simulink model "TAFC5B01"  (R2025b)
settings: Solver=ode4  StartTime=0.0  StopTime=inf  FixedStep=0.002  RelTol=1e-3
undefined symbols (not defined in the file): RS232, RS422, TTL, UART4, UART5, UART6, UART7, UART8
libraries: AFCToolbox x62, AFC5Toolbox x12, etargetslib x10, simulink x5
settings Model: Creator=Administrator  LastModifiedBy=zqhkd
settings OptimizationCC: DefaultParameterBehavior=Inlined  EnhancedBackFolding=on  PassReuseOutputArgsAs=Individual arguments  ZeroExternalMemoryAtStartup=off  ZeroInternalMemoryAtStartup=off  OptimizeBlockOrder=speed  DifferentSizesBufferReuse=on  OptimizationCustomize=off  EfficientTunableParamExpr=on
settings DebuggingCC: ParameterPrecisionLossMsg=none  ParameterTunabilityLossMsg=error
settings HardwareCC: ProdBitPerInt=16.0  ProdBitPerPointer=16.0  ProdBitPerSizeT=16.0  ProdBitPerPtrDiffT=16.0  ProdLargestAtomicFloat=None  ProdWordSize=16.0  ProdHWDeviceType=STMicroelectronics->ST10/Super10
settings SFSimCC: MATLABDynamicMemAlloc=off
settings RTWCC: SystemTargetFile=AFCHawk.tlc  GenCodeOnly=on  TemplateMakefile=ert_default_tmf  GPUComputeCapability=3.5  Description=Embedded Coder
settings CodeAppCC: ForceParamTrailComments=on  IgnoreCustomStorageClasses=off  OperatorAnnotations=on  SimulinkDataObjDesc=on  SFDataObjDesc=on  InsertBlockDesc=on
settings STFCustomTargetCC: SystemTargetFile=AFCHawk.tlc  TargetLangStandard=C99 (ISO)  MultiwordLength=256.0  ModelReferenceCompliant=off  ConcurrentExecutionCompliant=off  CombineOutputUpdateFcns=on  ERTCustomFileBanners=on  SupportContinuousTime=off  SupportNonInlinedSFcns=off  RemoveResetFunc=on  MATLABClassNameForMDSCustomization=Simulink.SoftwareTarget.ERTCustomization  GRTInterface=off  t_comBaud=460800.0  t_comPort=2.0  t_BuildCPrj2Hex=on  t_DownLoad2Target=on
settings ERTTargetCC: ERTCustomFileTemplate=example_file_process.tlc  DynamicArrayContainerType=coder::array  TargetLangStandard=C99 (ISO)  ModelReferenceCompliant=off  ParMdlRefBuildCompliant=off  CompOptLevelCompliant=off  ConcurrentExecutionCompliant=off  ModelStepFunctionPrototypeControlCompliant=off  CPPClassGenCompliant=off  UseToolchainInfoCompliant=off

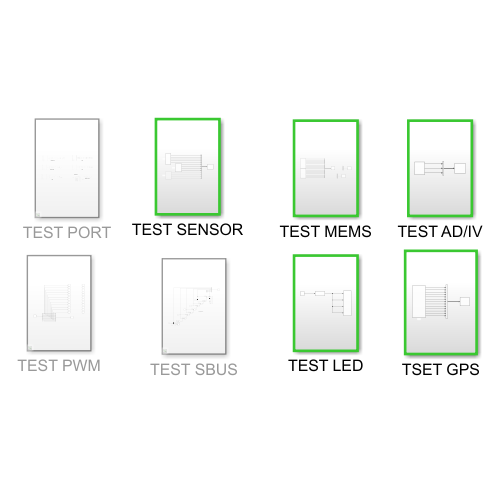
[thumbnail: Simulink's stored preview of the top-level diagram]
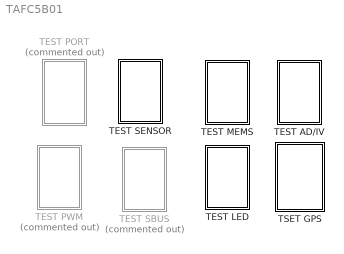
== system TAFC5B01 ==
  TEST AD/IV : Subsystem
  TEST LED : Subsystem
  TEST MEMS : Subsystem
  TEST PORT : Subsystem  Commented=on
  TEST PWM : Subsystem  Commented=on
  TEST SBUS : Subsystem  Commented=on
  TEST SENSOR : Subsystem
  TSET GPS : Subsystem

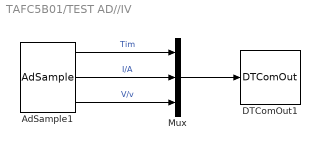
== system TAFC5B01/TEST AD//IV ==
  AdSample1 : AFCToolbox/DeviceModule/AdSample  Priority=1  g_sampleTime=0.01  g_comPort=0  g_instName=0  g_id=0
      settings: SourceProductName=AFCToolbox
  DTComOut1 : AFCToolbox/DeviceModule/DTComOut  Priority=8  g_frameType=12  g_outFreq=1  g_comPort=0  g_instName=0  g_id=0
      settings: SourceProductName=AFCToolbox
  Mux : Mux  Inputs=3
  wires:
  Mux/1 -> DTComOut1/1
  AdSample1/1 -> Mux/1  "Tim"
  AdSample1/2 -> Mux/2  "I/A"
  AdSample1/3 -> Mux/3  "V/v"

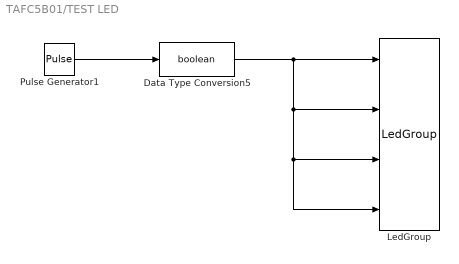
== system TAFC5B01/TEST LED ==
  Data Type Conversion5 : DataTypeConversion  OutDataTypeStr=boolean  SaturateOnIntegerOverflow=off  RndMeth=Floor
  LedGroup : AFCToolbox/DeviceModule/LedGroup  Priority=7  g_frameType=0  g_comPort=6  g_instName=0  g_id=0
      settings: SourceProductName=AFCToolbox
  Pulse Generator1 : DiscretePulseGenerator  Period=100  PulseWidth=50  SampleTime=0.01
  wires:
  Data Type Conversion5/1 -> LedGroup/2, LedGroup/4, LedGroup/3, LedGroup/1
  Pulse Generator1/1 -> Data Type Conversion5/1

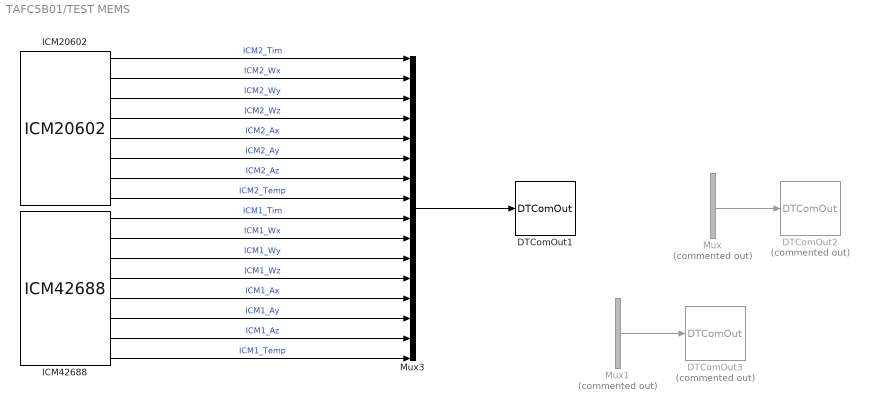
== system TAFC5B01/TEST MEMS ==
  DTComOut1 : AFCToolbox/DeviceModule/DTComOut  Priority=8  g_frameType=3  g_outFreq=10  g_comPort=0  g_instName=0  g_id=0
      settings: SourceProductName=AFCToolbox
  DTComOut2 : AFCToolbox/DeviceModule/DTComOut  Priority=8  Commented=on  g_frameType=1  g_outFreq=1  g_comPort=0  g_instName=0  g_id=0
      settings: SourceProductName=AFCToolbox
  DTComOut3 : AFCToolbox/DeviceModule/DTComOut  Priority=8  Commented=on  g_frameType=2  g_outFreq=1  g_comPort=0  g_instName=0  g_id=0
      settings: SourceProductName=AFCToolbox
  ICM20602 : AFCToolbox/DeviceModule/ICM20602  Priority=0  g_sampleTime=0.01  g_comPort=6  g_instName=0  g_id=0
      settings: SourceProductName=AFCToolbox
  ICM42688 : AFCToolbox/DeviceModule/ICM42688  Priority=0  g_sampleTime=0.01  g_comPort=6  g_instName=0  g_id=0
      settings: SourceProductName=AFCToolbox
  Mux : Mux  Commented=on  Inputs=14
  Mux1 : Mux  Commented=on  Inputs=15
  Mux3 : Mux  Inputs=16
  wires:
  ICM20602/4 -> Mux3/4  "ICM2_Wz"
  Mux3/1 -> DTComOut1/1
  ICM20602/6 -> Mux3/6  "ICM2_Ay"
  ICM42688/7 -> Mux3/15  "ICM1_Az"
  ICM42688/3 -> Mux3/11  "ICM1_Wy"
  ICM20602/3 -> Mux3/3  "ICM2_Wy"
  ICM20602/1 -> Mux3/1  "ICM2_Tim"
  ICM20602/2 -> Mux3/2  "ICM2_Wx"
  ICM20602/8 -> Mux3/8  "ICM2_Temp"
  ICM20602/7 -> Mux3/7  "ICM2_Az"
  ICM42688/1 -> Mux3/9  "ICM1_Tim"
  ICM42688/4 -> Mux3/12  "ICM1_Wz"
  ICM42688/2 -> Mux3/10  "ICM1_Wx"
  ICM20602/5 -> Mux3/5  "ICM2_Ax"
  ICM42688/5 -> Mux3/13  "ICM1_Ax"
  ICM42688/6 -> Mux3/14  "ICM1_Ay"
  ICM42688/8 -> Mux3/16  "ICM1_Temp"
  Mux/1 -> DTComOut2/1
  Mux1/1 -> DTComOut3/1

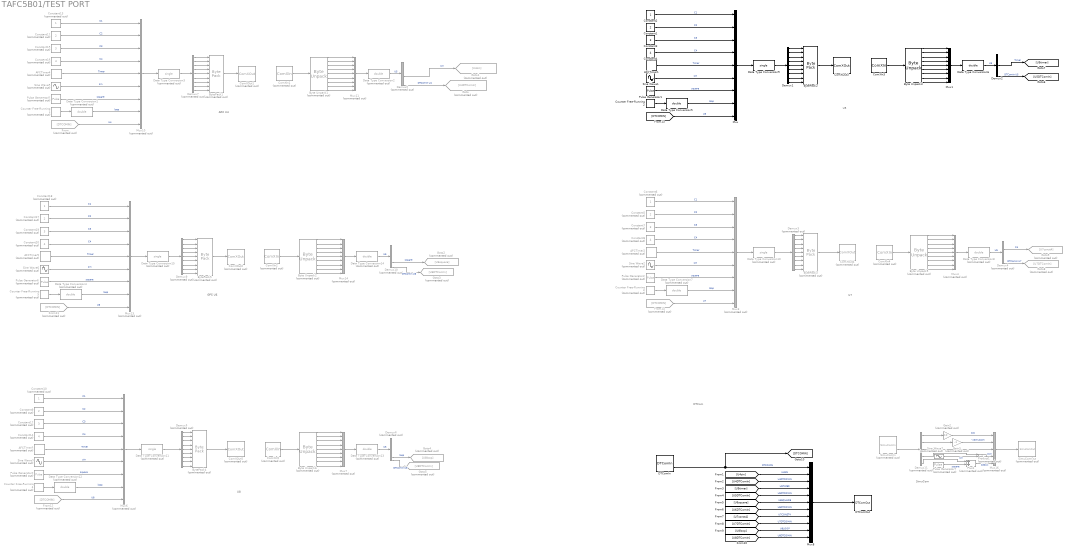
== system TAFC5B01/TEST PORT ==
  note: U5
  note: U7
  note: U8
  note: DTCom
  note: AGX U4
  note: GPS U6
  note: SimuCom
  AFCTimer1 : AFCToolbox/DeviceModule/AFCTimer  Priority=0  g_sampleTime=0.01  g_comPort=6  g_instName=0  g_id=0
      settings: SourceProductName=AFCToolbox
  AFCTimer{2..5} (4 alike) : AFCToolbox/DeviceModule/AFCTimer  Priority=0  Commented=on  g_sampleTime=0.01  g_comPort=6  g_instName=0  g_id=0
      settings: SourceProductName=AFCToolbox
  Byte Unpack{1..2,5..6} (4 alike) : etargetslib/Byte Unpack  Commented=on  dimensions={1,1,1,1,1,1,1,1,1}  datatypes={'single','single','single','single','single','single','single','single','single'}  byteAlign=1
      settings: LibrarySourceBlock=embeddedtargetslib/Host Communication/Byte Unpack
  Byte Unpack3 : etargetslib/Byte Unpack  dimensions={1,1,1,1,1,1,1,1,1}  datatypes={'single','single','single','single','single','single','single','single','single'}  byteAlign=1
      settings: LibrarySourceBlock=embeddedtargetslib/Host Communication/Byte Unpack
  BytePack{1,3..5} (4 alike) : etargetslib/Byte Pack  Commented=on  datatypes={'single','single','single','single','single','single','single','single','single'}  byteAlign=1
  BytePack2 : etargetslib/Byte Pack  datatypes={'single','single','single','single','single','single','single','single','single'}  byteAlign=1
  ComXIn1 : AFCToolbox/DeviceModule/ComXIn  Priority=2  Commented=on  g_sampleTime=0.01  g_comPort=UART4(TTL)  g_baudRate=460800  g_dataSize=36  g_parity=0  g_stopBits=1
      settings: SourceProductName=AFCToolbox
  ComXIn2 : AFCToolbox/DeviceModule/ComXIn  Priority=2  Commented=on  g_sampleTime=0.01  g_comPort=UART6(TTL)  g_baudRate=460800  g_dataSize=36  g_parity=0  g_stopBits=1
      settings: SourceProductName=AFCToolbox
  ComXIn3 : AFCToolbox/DeviceModule/ComXIn  Priority=2  g_sampleTime=0.01  g_comPort=UART5(RS422)  g_baudRate=460800  g_dataSize=36  g_parity=0  g_stopBits=1
      settings: SourceProductName=AFCToolbox
  ComXIn4 : AFCToolbox/DeviceModule/ComXIn  Priority=2  Commented=on  g_sampleTime=0.01  g_comPort=UART7(RS232)  g_baudRate=460800  g_dataSize=36  g_parity=0  g_stopBits=1
      settings: SourceProductName=AFCToolbox
  ComXIn5 : AFCToolbox/DeviceModule/ComXIn  Priority=2  Commented=on  g_sampleTime=0.01  g_comPort=UART8(RS232)  g_baudRate=460800  g_dataSize=36  g_parity=0  g_stopBits=1
      settings: SourceProductName=AFCToolbox
  ComXOut1 : AFCToolbox/DeviceModule/ComXOut  Priority=8  Commented=on  g_comPort=UART4(TTL)  g_baudRate=460800  g_outFreq=10
      settings: SourceProductName=AFCToolbox
  ComXOut2 : AFCToolbox/DeviceModule/ComXOut  Priority=8  Commented=on  g_comPort=UART6(TTL)  g_baudRate=460800  g_outFreq=10
      settings: SourceProductName=AFCToolbox
  ComXOut3 : AFCToolbox/DeviceModule/ComXOut  Priority=8  g_comPort=UART5(RS422)  g_baudRate=460800  g_outFreq=10
      settings: SourceProductName=AFCToolbox
  ComXOut4 : AFCToolbox/DeviceModule/ComXOut  Priority=8  Commented=on  g_comPort=UART7(RS232)  g_baudRate=460800  g_outFreq=10
      settings: SourceProductName=AFCToolbox
  ComXOut5 : AFCToolbox/DeviceModule/ComXOut  Priority=8  Commented=on  g_comPort=UART8(RS232)  g_baudRate=460800  g_outFreq=10
      settings: SourceProductName=AFCToolbox
  Constant1 : Constant  Value=2
  Constant{6,10,13,18} (4 alike) : Constant  Commented=on
  Constant{5,9,11,17} (4 alike) : Constant  Commented=on  Value=2
  Constant{7,12,15,19} (4 alike) : Constant  Commented=on  Value=3
  Constant{8,14,16,20} (4 alike) : Constant  Commented=on  Value=4
  Constant2 : Constant
  Constant3 : Constant  Value=3
  Constant4 : Constant  Value=4
  Counter Free-Running{1,3..5} (4 alike) : simulink/Sources/Counter Free-Running  Commented=on  NumBits=8  tsamp=-1
  Counter Free-Running2 : simulink/Sources/Counter Free-Running  NumBits=8  tsamp=-1
  DTComIn : AFCToolbox/DeviceModule/DTComIn  Priority=2  g_sampleTime=0.01  g_frameType=22  g_resFrameNum=0  g_comPort=6  g_instName=0  g_id=0
      settings: SourceProductName=AFCToolbox
  DTComOut : AFCToolbox/DeviceModule/DTComOut  Priority=8  g_frameType=21  g_outFreq=1  g_comPort=0  g_instName=0  g_id=0
      settings: SourceProductName=AFCToolbox
  Data Type Conversion{1..2,4,7..8,12..14} (8 alike) : DataTypeConversion  Commented=on  OutDataTypeStr=double  SaturateOnIntegerOverflow=off  RndMeth=Floor
  Data Type Conversion{3,10..11,15} (4 alike) : DataTypeConversion  Commented=on  OutDataTypeStr=single  SaturateOnIntegerOverflow=off  RndMeth=Floor
  Data Type Conversion5 : DataTypeConversion  OutDataTypeStr=double  SaturateOnIntegerOverflow=off  RndMeth=Floor
  Data Type Conversion6 : DataTypeConversion  OutDataTypeStr=double  SaturateOnIntegerOverflow=off  RndMeth=Floor
  Data Type Conversion9 : DataTypeConversion  OutDataTypeStr=single  SaturateOnIntegerOverflow=off  RndMeth=Floor
  Demux1 : Demux  Outputs=9
  Demux{3..10} (8 alike) : Demux  Commented=on  Outputs=9
  Demux11 : Demux  Commented=on  Outputs=5
  Demux2 : Demux  Outputs=9
  From{,11..12,14} (4 alike) : From  Commented=on  GotoTag=DTCOMIN
  Gain2 : Gain  Commented=on  Gain=10
  Gain3 : Gain  Commented=on  Gain=-1
  Goto : Goto  Commented=on  GotoTag=U4DTComIn
  Goto1 : Goto  Commented=on  GotoTag=U4sin
  Goto2 : Goto  Commented=on  GotoTag=U6square
  Goto3 : Goto  Commented=on  GotoTag=U6DTComIn
  Goto4 : Goto  Commented=on  GotoTag=U8loop
  Goto5 : Goto  Commented=on  GotoTag=U8DTComIn
  Goto8 : Goto  Commented=on  GotoTag=U7DTComIn
  Goto9 : Goto  Commented=on  GotoTag=U7const4
  Mux : Mux  Inputs=9
  Mux1 : Mux  Inputs=9
  Mux{3..4,6..7,10..11,13..14} (8 alike) : Mux  Commented=on  Inputs=9
  Mux16 : Mux  Commented=on  Inputs=5
  Mux8 : Mux  Inputs=11
  Plus1 : Sum  Commented=on
  Product1 : Product  Commented=on
  Pulse Generator1 : DiscretePulseGenerator  PulseType=Time based  Amplitude=100  Period=1  PulseWidth=50
  Pulse Generator{2..3,5..7} (5 alike) : DiscretePulseGenerator  Commented=on  PulseType=Time based  Amplitude=100  Period=1  PulseWidth=50
  SimuComIn : AFCToolbox/DeviceModule/SimuComIn  Priority=2  Commented=on  g_sampleTime=0.01  g_frameType=81  g_resFrameNum=0  g_comPort=6  g_instName=0  g_id=0
      settings: SourceProductName=AFCToolbox
  SimuComOut : AFCToolbox/DeviceModule/SimuComOut  Priority=8  Commented=on  g_frameType=1  g_outFreq=1  g_comPort=0  g_instName=0  g_id=0
      settings: SourceProductName=AFCToolbox
  Sine Wave1 : Sin  SineType=Sample based  Samples=100  SampleTime=0.01
  Sine Wave{2..3,5..7} (5 alike) : Sin  Commented=on  SineType=Sample based  Samples=100  SampleTime=0.01
  wires:
  AFCTimer1/1 -> Mux/5  "Timer"
  Data Type Conversion5/1 -> Mux/8  "loop"
  Constant2/1 -> Mux/1  "C1"
  Counter Free-Running2/1 -> Data Type Conversion5/1
  Pulse Generator1/1 -> Mux/7  "square"
  Sine Wave1/1 -> Mux/6  "sin"
  Constant4/1 -> Mux/4  "C4"
  Constant3/1 -> Mux/3  "C3"
  Constant1/1 -> Mux/2  "C2"
  [DTCOMIN] -> Mux/9  "U5"
  Demux1/1 -> BytePack2/1
  Demux1/2 -> BytePack2/2
  Demux1/3 -> BytePack2/3
  Demux1/4 -> BytePack2/4
  Demux1/5 -> BytePack2/5
  Demux1/6 -> BytePack2/6
  Demux1/7 -> BytePack2/7
  Demux1/8 -> BytePack2/8
  Demux1/9 -> BytePack2/9
  Mux/1 -> Data Type Conversion9/1
  BytePack2/1 -> ComXOut3/1
  ComXIn3/1 -> Byte Unpack3/1
  Byte Unpack3/1 -> Mux1/1
  Byte Unpack3/2 -> Mux1/2
  Byte Unpack3/3 -> Mux1/3
  Byte Unpack3/4 -> Mux1/4
  Byte Unpack3/5 -> Mux1/5
  Byte Unpack3/6 -> Mux1/6
  Byte Unpack3/7 -> Mux1/7
  Byte Unpack3/8 -> Mux1/8
  Byte Unpack3/9 -> Mux1/9
  Mux1/1 -> Data Type Conversion6/1
  Data Type Conversion6/1 -> Demux2/1  "U5"
  ComXIn4/1 -> Byte Unpack5/1
  Demux3/9 -> BytePack3/9
  Demux3/4 -> BytePack3/4
  Demux3/3 -> BytePack3/3
  Demux3/2 -> BytePack3/2
  BytePack3/1 -> ComXOut4/1
  Mux3/1 -> Data Type Conversion10/1
  Counter Free-Running3/1 -> Data Type Conversion7/1
  From14/1 -> Mux3/9  "U7"
  Demux3/6 -> BytePack3/6
  Demux3/7 -> BytePack3/7
  Sine Wave2/1 -> Mux3/6  "sin"
  Demux3/8 -> BytePack3/8
  AFCTimer2/1 -> Mux3/5  "Timer"
  Constant5/1 -> Mux3/2  "C2"
  Constant6/1 -> Mux3/1  "C1"
  Constant8/1 -> Mux3/4  "C4"
  Data Type Conversion7/1 -> Mux3/8  "loop"
  Demux3/5 -> BytePack3/5
  Constant7/1 -> Mux3/3  "C3"
  Byte Unpack5/7 -> Mux4/7
  Pulse Generator2/1 -> Mux3/7  "square"
  Data Type Conversion8/1 -> Demux4/1  "U5"
  Byte Unpack5/9 -> Mux4/9
  Byte Unpack5/2 -> Mux4/2
  Byte Unpack5/6 -> Mux4/6
  Demux3/1 -> BytePack3/1
  Byte Unpack5/3 -> Mux4/3
  Mux4/1 -> Data Type Conversion8/1
  Byte Unpack5/5 -> Mux4/5
  Byte Unpack5/4 -> Mux4/4
  Byte Unpack5/1 -> Mux4/1
  Byte Unpack5/8 -> Mux4/8
  Data Type Conversion9/1 -> Demux1/1
  Data Type Conversion10/1 -> Demux3/1
  Data Type Conversion11/1 -> Demux5/1
  Data Type Conversion13/1 -> Demux6/1  "U5"
  Data Type Conversion12/1 -> Mux6/8  "loop"
  Demux5/5 -> BytePack4/5
  Byte Unpack6/9 -> Mux7/9
  Pulse Generator3/1 -> Mux6/7  "square"
  Constant9/1 -> Mux6/2  "C2"
  From12/1 -> Mux6/9  "U8"
  Demux5/8 -> BytePack4/8
  Sine Wave3/1 -> Mux6/6  "sin"
  Demux5/3 -> BytePack4/3
  Demux5/2 -> BytePack4/2
  Mux6/1 -> Data Type Conversion11/1
  Demux5/6 -> BytePack4/6
  Demux5/9 -> BytePack4/9
  AFCTimer3/1 -> Mux6/5  "Timer"
  BytePack4/1 -> ComXOut5/1
  Byte Unpack6/7 -> Mux7/7
  Constant12/1 -> Mux6/3  "C3"
  Byte Unpack6/2 -> Mux7/2
  ComXIn5/1 -> Byte Unpack6/1
  Demux5/4 -> BytePack4/4
  Constant14/1 -> Mux6/4  "C4"
  Byte Unpack6/5 -> Mux7/5
  Byte Unpack6/6 -> Mux7/6
  Byte Unpack6/8 -> Mux7/8
  Byte Unpack6/4 -> Mux7/4
  Counter Free-Running4/1 -> Data Type Conversion12/1
  Mux7/1 -> Data Type Conversion13/1
  Demux5/1 -> BytePack4/1
  Constant10/1 -> Mux6/1  "C1"
  Byte Unpack6/3 -> Mux7/3
  Demux5/7 -> BytePack4/7
  Byte Unpack6/1 -> Mux7/1
  Mux8/1 -> DTComOut/1
  Byte Unpack1/1 -> Mux11/1
  Byte Unpack1/9 -> Mux11/9
  Byte Unpack1/2 -> Mux11/2
  AFCTimer4/1 -> Mux10/5  "Timer"
  Demux7/8 -> BytePack1/8
  Counter Free-Running1/1 -> Data Type Conversion1/1
  Demux7/5 -> BytePack1/5
  Data Type Conversion3/1 -> Demux7/1
  Data Type Conversion1/1 -> Mux10/8  "loop"
  Byte Unpack1/3 -> Mux11/3
  Byte Unpack1/6 -> Mux11/6
  Demux7/4 -> BytePack1/4
  Byte Unpack1/4 -> Mux11/4
  Constant15/1 -> Mux10/3  "C3"
  Mux11/1 -> Data Type Conversion2/1
  Byte Unpack1/7 -> Mux11/7
  Data Type Conversion2/1 -> Demux8/1  "U5"
  Constant11/1 -> Mux10/2  "C2"
  Demux7/7 -> BytePack1/7
  Demux7/2 -> BytePack1/2
  Byte Unpack1/5 -> Mux11/5
  Mux10/1 -> Data Type Conversion3/1
  Demux7/1 -> BytePack1/1
  Demux7/9 -> BytePack1/9
  Demux7/6 -> BytePack1/6
  Byte Unpack1/8 -> Mux11/8
  Sine Wave5/1 -> Mux10/6  "sin"
  Pulse Generator5/1 -> Mux10/7  "square"
  Demux7/3 -> BytePack1/3
  Constant13/1 -> Mux10/1  "C1"
  Constant16/1 -> Mux10/4  "C4"
  BytePack1/1 -> ComXOut1/1
  ComXIn1/1 -> Byte Unpack1/1
  Constant20/1 -> Mux13/4  "C4"
  Sine Wave6/1 -> Mux13/6  "sin"
  Demux9/3 -> BytePack5/3
  Demux9/7 -> BytePack5/7
  Demux9/6 -> BytePack5/6
  Demux9/9 -> BytePack5/9
  Mux13/1 -> Data Type Conversion15/1
  Byte Unpack2/5 -> Mux14/5
  Byte Unpack2/8 -> Mux14/8
  Constant17/1 -> Mux13/2  "C2"
  Data Type Conversion14/1 -> Demux10/1  "U5"
  Constant18/1 -> Mux13/1  "C1"
  Demux9/1 -> BytePack5/1
  From11/1 -> Mux13/9  "U6"
  Demux9/4 -> BytePack5/4
  Constant19/1 -> Mux13/3  "C3"
  Byte Unpack2/4 -> Mux14/4
  Byte Unpack2/6 -> Mux14/6
  Byte Unpack2/7 -> Mux14/7
  Data Type Conversion4/1 -> Mux13/8  "loop"
  Mux14/1 -> Data Type Conversion14/1
  Byte Unpack2/3 -> Mux14/3
  Pulse Generator6/1 -> Mux13/7  "square"
  Byte Unpack2/2 -> Mux14/2
  Demux9/8 -> BytePack5/8
  AFCTimer5/1 -> Mux13/5  "Timer"
  Demux9/5 -> BytePack5/5
  Byte Unpack2/9 -> Mux14/9
  Data Type Conversion15/1 -> Demux9/1
  Byte Unpack2/1 -> Mux14/1
  Demux9/2 -> BytePack5/2
  Counter Free-Running5/1 -> Data Type Conversion4/1
  BytePack5/1 -> ComXOut2/1
  ComXIn2/1 -> Byte Unpack2/1
  Demux11/4 -> Product1/1
  Plus1/1 -> Mux16/5  "100x/x"
  SimuComIn/2 -> Demux11/1
  Product1/1 -> Mux16/4  "xsin"
  Pulse Generator7/1 -> Plus1/2  "square"
  Gain3/1 -> Mux16/2  "-xSimuCom"
  Mux16/1 -> SimuComOut/1
  Demux11/5 -> Plus1/1
  Demux11/3 -> Mux16/3
  Sine Wave7/1 -> Product1/2  "sin"
  Demux11/2 -> Gain3/1
  Demux11/1 -> Gain2/1
  Gain2/1 -> Mux16/1  "10x"
  Demux8/9 -> Goto/1  "DTComIn U4"
  [U4DTComIn] -> Mux8/3  "U4DTCOMIN"
  Demux8/6 -> Goto1/1  "sin"
  [U4sin] -> Mux8/2  "U4SIN"
  Demux10/7 -> Goto2/1  "square"
  Demux10/9 -> Goto3/1  "DTComIn U6"
  Demux6/8 -> Goto4/1  "loop"
  Demux6/9 -> Goto5/1  "DTComIn U8"
  Demux2/9 -> [U5DTComIn]  "DTComIn U5"
  Demux2/5 -> [U5timer]  "Timer"
  Demux4/9 -> Goto8/1  "DTComIn U7"
  Demux4/4 -> Goto9/1  "C4"
  [U5timer] -> Mux8/4  "U5TIMER"
  [U5DTComIn] -> Mux8/5  "U5DTCOMIN"
  [U6square] -> Mux8/6  "U6SQUARE"
  [U6DTComIn] -> Mux8/7  "U6DTCOMIN"
  [U7const4] -> Mux8/8  "U7CONST4"
  [U7DTComIn] -> Mux8/9  "U7DTCOMIN"
  [U8loop] -> Mux8/10  "U8LOOP"
  [U8DTComIn] -> Mux8/11  "U8DTCOMIN"
  DTComIn/2 -> [DTCOMIN], Mux8/1  "DTCOMIN"
  From/1 -> Mux10/9  "U4"

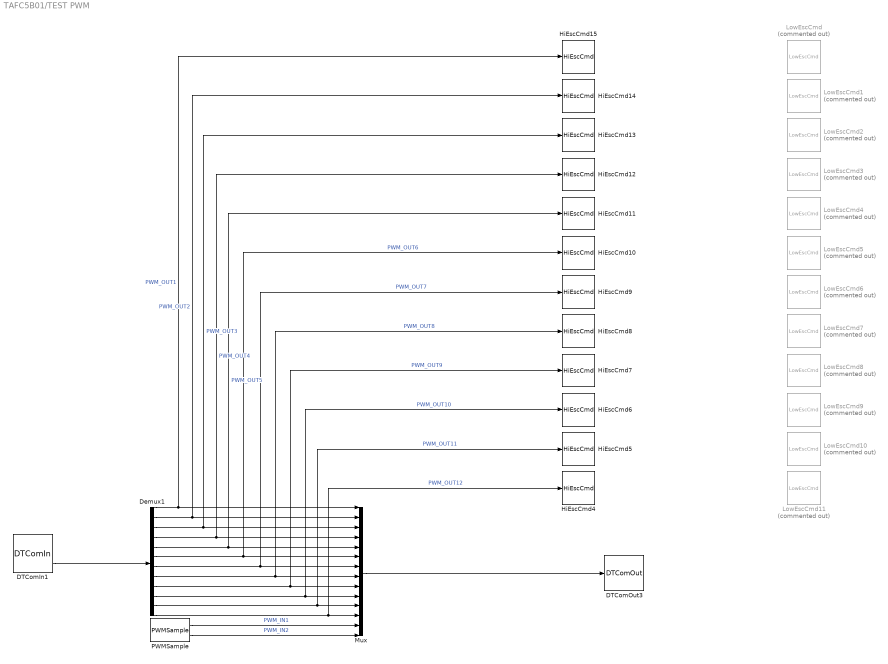
== system TAFC5B01/TEST PWM ==
  DTComIn1 : AFCToolbox/DeviceModule/DTComIn  Priority=2  g_sampleTime=0.01  g_frameType=44  g_resFrameNum=0  g_comPort=6  g_instName=0  g_id=0
      settings: SourceProductName=AFCToolbox
  DTComOut3 : AFCToolbox/DeviceModule/DTComOut  Priority=8  g_frameType=14  g_outFreq=10  g_comPort=0  g_instName=0  g_id=0
      settings: SourceProductName=AFCToolbox
  Demux1 : Demux  Outputs=12
  HiEscCmd10 : AFCToolbox/DeviceModule/HiEscCmd  Priority=6  g_chanelNo=6  g_minPW=0  g_maxPW=100  g_comPort=6  g_instName=0  g_id=0
      settings: SourceProductName=AFCToolbox
  HiEscCmd11 : AFCToolbox/DeviceModule/HiEscCmd  Priority=6  g_chanelNo=5  g_minPW=0  g_maxPW=100  g_comPort=6  g_instName=0  g_id=0
      settings: SourceProductName=AFCToolbox
  HiEscCmd12 : AFCToolbox/DeviceModule/HiEscCmd  Priority=6  g_chanelNo=4  g_minPW=0  g_maxPW=100  g_comPort=6  g_instName=0  g_id=0
      settings: SourceProductName=AFCToolbox
  HiEscCmd13 : AFCToolbox/DeviceModule/HiEscCmd  Priority=6  g_chanelNo=3  g_minPW=0  g_maxPW=100  g_comPort=6  g_instName=0  g_id=0
      settings: SourceProductName=AFCToolbox
  HiEscCmd14 : AFCToolbox/DeviceModule/HiEscCmd  Priority=6  g_chanelNo=2  g_minPW=0  g_maxPW=100  g_comPort=6  g_instName=0  g_id=0
      settings: SourceProductName=AFCToolbox
  HiEscCmd15 : AFCToolbox/DeviceModule/HiEscCmd  Priority=6  g_chanelNo=1  g_minPW=0  g_maxPW=100  g_comPort=6  g_instName=0  g_id=0
      settings: SourceProductName=AFCToolbox
  HiEscCmd4 : AFCToolbox/DeviceModule/HiEscCmd  Priority=6  g_chanelNo=12  g_minPW=0  g_maxPW=100  g_comPort=6  g_instName=0  g_id=0
      settings: SourceProductName=AFCToolbox
  HiEscCmd5 : AFCToolbox/DeviceModule/HiEscCmd  Priority=6  g_chanelNo=11  g_minPW=0  g_maxPW=100  g_comPort=6  g_instName=0  g_id=0
      settings: SourceProductName=AFCToolbox
  HiEscCmd6 : AFCToolbox/DeviceModule/HiEscCmd  Priority=6  g_chanelNo=10  g_minPW=0  g_maxPW=100  g_comPort=6  g_instName=0  g_id=0
      settings: SourceProductName=AFCToolbox
  HiEscCmd7 : AFCToolbox/DeviceModule/HiEscCmd  Priority=6  g_chanelNo=9  g_minPW=0  g_maxPW=100  g_comPort=6  g_instName=0  g_id=0
      settings: SourceProductName=AFCToolbox
  HiEscCmd8 : AFCToolbox/DeviceModule/HiEscCmd  Priority=6  g_chanelNo=8  g_minPW=0  g_maxPW=100  g_comPort=6  g_instName=0  g_id=0
      settings: SourceProductName=AFCToolbox
  HiEscCmd9 : AFCToolbox/DeviceModule/HiEscCmd  Priority=6  g_chanelNo=7  g_minPW=0  g_maxPW=100  g_comPort=6  g_instName=0  g_id=0
      settings: SourceProductName=AFCToolbox
  LowEscCmd : AFC5Toolbox/DeviceModule/LowEscCmd  Priority=6  Commented=on  g_chanelNo=1  g_minPW=0  g_maxPW=100  g_comPort=6  g_instName=0  g_id=0
  LowEscCmd1 : AFC5Toolbox/DeviceModule/LowEscCmd  Priority=6  Commented=on  g_chanelNo=2  g_minPW=0  g_maxPW=100  g_comPort=6  g_instName=0  g_id=0
  LowEscCmd10 : AFC5Toolbox/DeviceModule/LowEscCmd  Priority=6  Commented=on  g_chanelNo=11  g_minPW=0  g_maxPW=100  g_comPort=6  g_instName=0  g_id=0
  LowEscCmd11 : AFC5Toolbox/DeviceModule/LowEscCmd  Priority=6  Commented=on  g_chanelNo=12  g_minPW=0  g_maxPW=100  g_comPort=6  g_instName=0  g_id=0
  LowEscCmd2 : AFC5Toolbox/DeviceModule/LowEscCmd  Priority=6  Commented=on  g_chanelNo=3  g_minPW=0  g_maxPW=100  g_comPort=6  g_instName=0  g_id=0
  LowEscCmd3 : AFC5Toolbox/DeviceModule/LowEscCmd  Priority=6  Commented=on  g_chanelNo=4  g_minPW=0  g_maxPW=100  g_comPort=6  g_instName=0  g_id=0
  LowEscCmd4 : AFC5Toolbox/DeviceModule/LowEscCmd  Priority=6  Commented=on  g_chanelNo=5  g_minPW=0  g_maxPW=100  g_comPort=6  g_instName=0  g_id=0
  LowEscCmd5 : AFC5Toolbox/DeviceModule/LowEscCmd  Priority=6  Commented=on  g_chanelNo=6  g_minPW=0  g_maxPW=100  g_comPort=6  g_instName=0  g_id=0
  LowEscCmd6 : AFC5Toolbox/DeviceModule/LowEscCmd  Priority=6  Commented=on  g_chanelNo=7  g_minPW=0  g_maxPW=100  g_comPort=6  g_instName=0  g_id=0
  LowEscCmd7 : AFC5Toolbox/DeviceModule/LowEscCmd  Priority=6  Commented=on  g_chanelNo=8  g_minPW=0  g_maxPW=100  g_comPort=6  g_instName=0  g_id=0
  LowEscCmd8 : AFC5Toolbox/DeviceModule/LowEscCmd  Priority=6  Commented=on  g_chanelNo=9  g_minPW=0  g_maxPW=100  g_comPort=6  g_instName=0  g_id=0
  LowEscCmd9 : AFC5Toolbox/DeviceModule/LowEscCmd  Priority=6  Commented=on  g_chanelNo=10  g_minPW=0  g_maxPW=100  g_comPort=6  g_instName=0  g_id=0
  Mux : Mux  Inputs=14
  PWMSample : AFCToolbox/DeviceModule/PWMSample  Priority=1  g_sampleTime=0.01  g_comPort=6  g_instName=0  g_id=0
      settings: SourceProductName=AFCToolbox
  wires:
  Demux1/3 -> HiEscCmd13/1, Mux/3  "PWM_OUT3"
  Demux1/10 -> HiEscCmd6/1, Mux/10  "PWM_OUT10"
  Demux1/8 -> HiEscCmd8/1, Mux/8  "PWM_OUT8"
  Demux1/11 -> HiEscCmd5/1, Mux/11  "PWM_OUT11"
  Demux1/1 -> HiEscCmd15/1, Mux/1  "PWM_OUT1"
  Demux1/5 -> HiEscCmd11/1, Mux/5  "PWM_OUT5"
  Demux1/7 -> HiEscCmd9/1, Mux/7  "PWM_OUT7"
  Demux1/12 -> HiEscCmd4/1, Mux/12  "PWM_OUT12"
  Mux/1 -> DTComOut3/1
  Demux1/6 -> HiEscCmd10/1, Mux/6  "PWM_OUT6"
  Demux1/9 -> HiEscCmd7/1, Mux/9  "PWM_OUT9"
  Demux1/2 -> HiEscCmd14/1, Mux/2  "PWM_OUT2"
  Demux1/4 -> HiEscCmd12/1, Mux/4  "PWM_OUT4"
  PWMSample/1 -> Mux/13  "PWM_IN1"
  PWMSample/2 -> Mux/14  "PWM_IN2"
  DTComIn1/2 -> Demux1/1

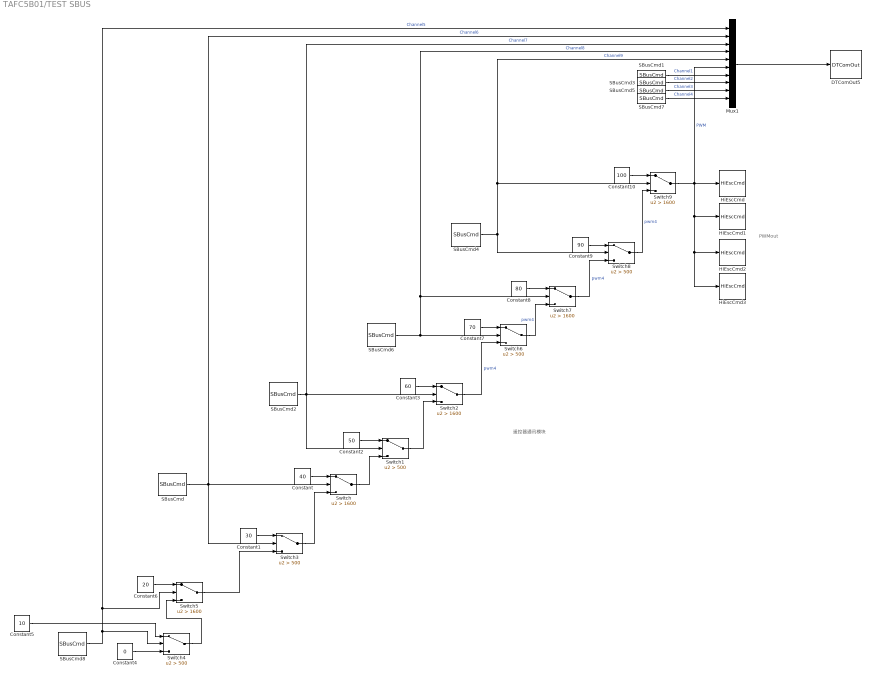
== system TAFC5B01/TEST SBUS ==
  note: 遥控器通讯模块
  note: PWMout
  Constant : Constant  Value=40
  Constant1 : Constant  Value=30
  Constant10 : Constant  Value=100
  Constant2 : Constant  Value=50
  Constant3 : Constant  Value=60
  Constant4 : Constant  Value=0
  Constant5 : Constant  Value=10
  Constant6 : Constant  Value=20
  Constant7 : Constant  Value=70
  Constant8 : Constant  Value=80
  Constant9 : Constant  Value=90
  DTComOut5 : AFCToolbox/DeviceModule/DTComOut  Priority=8  g_frameType=13  g_outFreq=10  g_comPort=0  g_instName=0  g_id=0
      settings: SourceProductName=AFCToolbox
  HiEscCmd : AFCToolbox/DeviceModule/HiEscCmd  Priority=6  g_chanelNo=1  g_minPW=40  g_maxPW=80  g_comPort=6  g_instName=0  g_id=0
      settings: SourceProductName=AFCToolbox
  HiEscCmd1 : AFCToolbox/DeviceModule/HiEscCmd  Priority=6  g_chanelNo=9  g_minPW=40  g_maxPW=80  g_comPort=6  g_instName=0  g_id=0
      settings: SourceProductName=AFCToolbox
  HiEscCmd2 : AFCToolbox/DeviceModule/HiEscCmd  Priority=6  g_chanelNo=7  g_minPW=40  g_maxPW=80  g_comPort=6  g_instName=0  g_id=0
      settings: SourceProductName=AFCToolbox
  HiEscCmd3 : AFCToolbox/DeviceModule/HiEscCmd  Priority=6  g_chanelNo=2  g_minPW=40  g_maxPW=80  g_comPort=6  g_instName=0  g_id=0
      settings: SourceProductName=AFCToolbox
  Mux1 : Mux  Inputs=10
  SBusCmd : AFCToolbox/DeviceModule/SBusCmd  Priority=0  g_sampleTime=0.01  g_chanelNo=6  g_comPort=6  g_instName=0  g_id=0
      settings: SourceProductName=AFCToolbox
  SBusCmd1 : AFCToolbox/DeviceModule/SBusCmd  Priority=0  g_sampleTime=0.01  g_chanelNo=1  g_comPort=6  g_instName=0  g_id=0
      settings: SourceProductName=AFCToolbox
  SBusCmd2 : AFCToolbox/DeviceModule/SBusCmd  Priority=0  g_sampleTime=0.01  g_chanelNo=7  g_comPort=6  g_instName=0  g_id=0
      settings: SourceProductName=AFCToolbox
  SBusCmd3 : AFCToolbox/DeviceModule/SBusCmd  Priority=0  g_sampleTime=0.01  g_chanelNo=2  g_comPort=6  g_instName=0  g_id=0
      settings: SourceProductName=AFCToolbox
  SBusCmd4 : AFCToolbox/DeviceModule/SBusCmd  Priority=0  g_sampleTime=0.01  g_chanelNo=9  g_comPort=6  g_instName=0  g_id=0
      settings: SourceProductName=AFCToolbox
  SBusCmd5 : AFCToolbox/DeviceModule/SBusCmd  Priority=0  g_sampleTime=0.01  g_chanelNo=3  g_comPort=6  g_instName=0  g_id=0
      settings: SourceProductName=AFCToolbox
  SBusCmd6 : AFCToolbox/DeviceModule/SBusCmd  Priority=0  g_sampleTime=0.01  g_chanelNo=8  g_comPort=6  g_instName=0  g_id=0
      settings: SourceProductName=AFCToolbox
  SBusCmd7 : AFCToolbox/DeviceModule/SBusCmd  Priority=0  g_sampleTime=0.01  g_chanelNo=4  g_comPort=6  g_instName=0  g_id=0
      settings: SourceProductName=AFCToolbox
  SBusCmd8 : AFCToolbox/DeviceModule/SBusCmd  Priority=0  g_sampleTime=0.01  g_chanelNo=5  g_comPort=6  g_instName=0  g_id=0
      settings: SourceProductName=AFCToolbox
  Switch{,2,5,7,9} (5 alike) : Switch  Criteria=u2 > Threshold  Threshold=1600  SaturateOnIntegerOverflow=off  InputSameDT=off
  Switch{1,3..4,6,8} (5 alike) : Switch  Criteria=u2 > Threshold  Threshold=500  SaturateOnIntegerOverflow=off  InputSameDT=off
  wires:
  Constant3/1 -> Switch2/1
  SBusCmd2/1 -> Mux1/3, Switch1/2, Switch2/2  "Channel7"
  Switch9/1 -> Mux1/6, HiEscCmd/1, HiEscCmd1/1, HiEscCmd3/1, HiEscCmd2/1  "PWM"
  SBusCmd8/1 -> Mux1/1, Switch5/2, Switch4/2  "Channel5"
  SBusCmd/1 -> Mux1/2, Switch/2, Switch3/2  "Channel6"
  Constant7/1 -> Switch6/1
  Constant2/1 -> Switch1/1
  SBusCmd6/1 -> Mux1/4, Switch7/2, Switch6/2  "Channel8"
  Switch2/1 -> Switch6/3  "pwm4"
  Switch4/1 -> Switch5/3
  Constant10/1 -> Switch9/1
  Switch3/1 -> Switch/3
  Constant4/1 -> Switch4/3
  Switch6/1 -> Switch7/3  "pwm4"
  Constant/1 -> Switch/1
  Constant1/1 -> Switch3/1
  Mux1/1 -> DTComOut5/1
  Constant8/1 -> Switch7/1
  SBusCmd4/1 -> Mux1/5, Switch9/2, Switch8/2  "Channel9"
  Switch8/1 -> Switch9/3  "pwm4"
  Switch5/1 -> Switch3/3
  Constant9/1 -> Switch8/1
  Constant5/1 -> Switch4/1
  Switch1/1 -> Switch2/3
  Switch7/1 -> Switch8/3  "pwm4"
  Switch/1 -> Switch1/3
  Constant6/1 -> Switch5/1
  SBusCmd1/1 -> Mux1/7  "Channel1"
  SBusCmd3/1 -> Mux1/8  "Channel2"
  SBusCmd5/1 -> Mux1/9  "Channel3"
  SBusCmd7/1 -> Mux1/10  "Channel4"

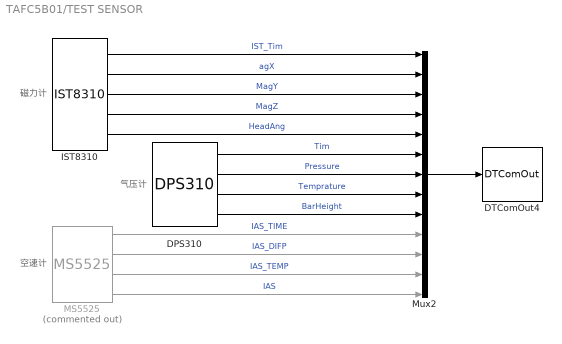
== system TAFC5B01/TEST SENSOR ==
  note: 空速计
  note: 磁力计
  note: 气压计
  DPS310 : AFCToolbox/DeviceModule/DPS310  Priority=1  g_sampleTime=0.01  g_comPort=6  g_instName=0  g_id=0
      settings: SourceProductName=AFCToolbox
  DTComOut4 : AFCToolbox/DeviceModule/DTComOut  Priority=8  g_frameType=2  g_outFreq=10  g_comPort=0  g_instName=0  g_id=0
      settings: SourceProductName=AFCToolbox
  IST8310 : AFCToolbox/DeviceModule/IST8310  Priority=1  g_sampleTime=0.01  g_comPort=0  g_instName=0  g_id=0
      settings: SourceProductName=AFCToolbox
  MS5525 : AFCToolbox/DeviceModule/MS5525  Priority=1  Commented=on  g_sampleTime=0.01  g_comPort=6  g_instName=0  g_id=0
      settings: SourceProductName=AFCToolbox
  Mux2 : Mux  Inputs=13
  wires:
  MS5525/3 -> Mux2/12  "IAS_TEMP"
  DPS310/3 -> Mux2/8  "Temprature"
  DPS310/1 -> Mux2/6  "Tim"
  IST8310/2 -> Mux2/2  "agX"
  MS5525/4 -> Mux2/13  "IAS"
  IST8310/4 -> Mux2/4  "MagZ"
  MS5525/2 -> Mux2/11  "IAS_DIFP"
  DPS310/4 -> Mux2/9  "BarHeight"
  DPS310/2 -> Mux2/7  "Pressure"
  IST8310/5 -> Mux2/5  "HeadAng"
  Mux2/1 -> DTComOut4/1
  IST8310/3 -> Mux2/3  "MagY"
  IST8310/1 -> Mux2/1  "IST_Tim"
  MS5525/1 -> Mux2/10  "IAS_TIME"

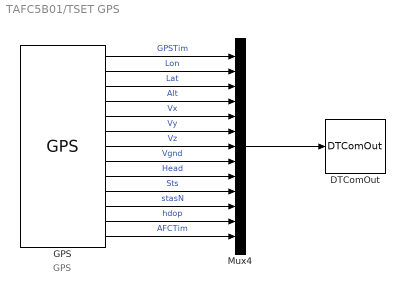
== system TAFC5B01/TSET GPS ==
  note: GPS
  DTComOut : AFCToolbox/DeviceModule/DTComOut  Priority=8  g_frameType=11  g_outFreq=1  g_comPort=0  g_instName=0  g_id=0
      settings: SourceProductName=AFCToolbox
  GPS : AFCToolbox/DeviceModule/GPS  Priority=1  g_sampleTime=0.01  g_gpsDev=M10 GNSS  g_comPort=6  g_instName=0  g_id=0
      settings: SourceProductName=AFCToolbox
  Mux4 : Mux  Inputs=13
  wires:
  GPS/3 -> Mux4/3  "Lat"
  GPS/13 -> Mux4/13  "AFCTim"
  GPS/1 -> Mux4/1  "GPSTim"
  GPS/10 -> Mux4/10  "Sts"
  GPS/9 -> Mux4/9  "Head"
  GPS/12 -> Mux4/12  "hdop"
  GPS/11 -> Mux4/11  "stasN"
  GPS/7 -> Mux4/7  "Vz"
  GPS/6 -> Mux4/6  "Vy"
  Mux4/1 -> DTComOut/1
  GPS/2 -> Mux4/2  "Lon"
  GPS/5 -> Mux4/5  "Vx"
  GPS/8 -> Mux4/8  "Vgnd"
  GPS/4 -> Mux4/4  "Alt"
